simulink model "Controller_implementacion"  (R2026a)
settings: Solver=FixedStepDiscrete  StopTime=inf  FixedStep=Ts  EnableMultiTasking=on
model workspace (MAT data in the model file):
  Ki_SIMC = Simulink.Parameter
  Ki_SIMC.Value = 0.079379
  Ki_SIMC.Complexity = 'real'
  Ki_SIMC.Dimensions = [1 1]
  Ki_SIMC.CoderInfo.StorageClass = 'ExportedGlobal'
  Ki_SIMC.DataType = 'auto'
  Kp_SIMC = Simulink.Parameter
  Kp_SIMC.Value = 7.620337
  Kp_SIMC.Complexity = 'real'
  Kp_SIMC.Dimensions = [1 1]
  Kp_SIMC.CoderInfo.StorageClass = 'ExportedGlobal'
  Kp_SIMC.DataType = 'auto'
  Q_max = Simulink.Parameter
  Q_max.Value = 90
  Q_max.Complexity = 'real'
  Q_max.Dimensions = [1 1]
  Q_max.CoderInfo.StorageClass = 'ExportedGlobal'
  Q_max.DataType = 'single'
  Q_min = Simulink.Parameter
  Q_min.Value = 0
  Q_min.Complexity = 'real'
  Q_min.Dimensions = [1 1]
  Q_min.CoderInfo.StorageClass = 'ExportedGlobal'
  Q_min.DataType = 'single'
  Ts = 1
libraries: slpidlib x1
settings Model: SILPILModeSetting=veronly  ExtModeTrigDuration=2  Creator=jguerrero  LastModifiedBy=jordy
settings HardwareCC: ProdBitPerInt=16.0  ProdBitPerPointer=16.0  ProdBitPerSizeT=16.0  ProdBitPerPtrDiffT=16.0  ProdWordSize=8.0  ProdHWDeviceType=Atmel->AVR
settings ModelReferenceCC: PropagateVarSize=During execution
settings RTWCC: SystemTargetFile=ert.tlc  HardwareBoard=Arduino Leonardo  TLCOptions=-aInlineSetEventsForThisBaseRateFcn=TLC_FALSE -aSuppressMultiTaskScheduler=TLC_FALSE -aRateBasedStepFcn=1  Toolchain=Arduino AVR  BuildConfiguration=Faster Runs  Description=Embedded Coder
settings ERTTargetCC: ExtModeTransport=3.0  ExtModeAutomaticAllocSize=off  ExtModeStaticAllocSize=250.0  CodeInterfacePackaging=Reusable function  SupportContinuousTime=on  SupportVariableSizeSignals=on

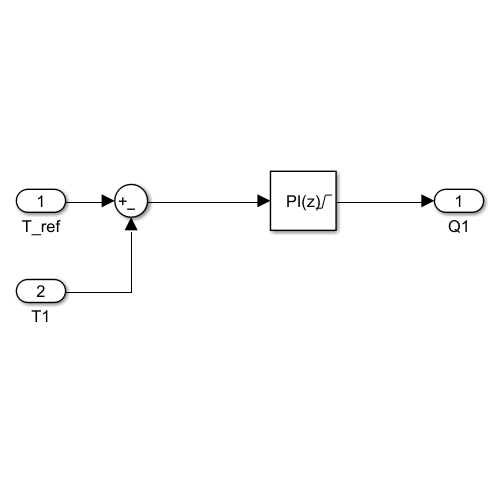
[thumbnail: Simulink's stored preview of the top-level diagram]
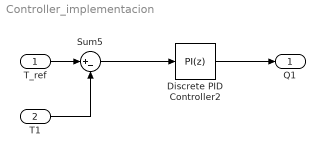
== system Controller_implementacion ==
  T_ref : Inport  OutDataTypeStr=single  PortDimensions=1  SampleTime=[1,0]
  T1 : Inport  Port=2  OutDataTypeStr=single  PortDimensions=1  SampleTime=[1,0]
  Discrete PID Controller2 : slpidlib/PID Controller  Controller=PI  Form=Parallel  TimeDomain=Discrete-time  UseExternalTs=off  SampleTime=Ts  IntegratorMethod=Forward Euler  FilterMethod=Forward Euler  ControllerParametersSource=internal  P=Kp_SIMC  I=Ki_SIMC  UseKiTs=off  D=0  UseExternalDerivativeSource=off  N=100  UseFilter=on  TunerSelectOption=Transfer Function Based (PID Tuner App)  InitialConditionSource=internal  InitialConditionForIntegrator=0  InitialConditionForFilter=0  DifferentiatorICPrevScaledInput=0  ExternalReset=none  TrackingMode=off  Kt=1  LimitOutput=on  SatLimitsSource=internal  UpperSaturationLimit=Q_max  LowerSaturationLimit=Q_min  LinearizeAsGain=off  AntiWindupMode=clamping  Kb=1  LimitIntegrator=off  UpperIntegratorSaturationLimit=inf  LowerIntegratorSaturationLimit=-inf  POutMin=[]  POutMax=[]  IOutMin=[]  IOutMax=[]  DOutMin=[]  DOutMax=[]  NOutMin=[]  NOutMax=[]  SumOutMin=[]  SumOutMax=[]  SaturationOutMin=[]  SaturationOutMax=[]  PParamMin=[]  PParamMax=[]  IParamMin=[]  IParamMax=[]  DParamMin=[]  DParamMax=[]  NParamMin=[]  NParamMax=[]  KbParamMin=[]  KbParamMax=[]  KtParamMin=[]  KtParamMax=[]  KbOutMin=[]  KbOutMax=[]  KtOutMin=[]  KtOutMax=[]  IntegratorOutMin=[]  IntegratorOutMax=[]  FilterOutMin=[]  FilterOutMax=[]  SumI1OutMin=[]  SumI1OutMax=[]  SumI2OutMin=[]  SumI2OutMax=[]  SumI3OutMin=[]  SumI3OutMax=[]  SumI4OutMin=[]  SumI4OutMax=[]  SumDOutMin=[]  SumDOutMax=[]  DifferentiatorOutMin=[]  DifferentiatorOutMax=[]  FilterDiffOutCoefMin=[]  FilterDiffOutCoefMax=[]  ReciprocalOutMin=[]  ReciprocalOutMax=[]  SumDenOutMin=[]  SumDenOutMax=[]  SumNumOutMin=[]  SumNumOutMax=[]  DivideOutMin=[]  DivideOutMax=[]  UdiffTsProdOutMin=[]  UdiffTsProdOutMax=[]  NTsProdOutMin=[]  NTsProdOutMax=[]  UintegralTsProdOutMin=[]  UintegralTsProdOutMax=[]  UngainTsProdOutMin=[]  UngainTsProdOutMax=[]  ClampingZeroOutDataTypeStr=Inherit: Inherit via back propagation  ClampingZeroOutMin=[]  ClampingZeroOutMax=[]  FilterDenConstantOutDataTypeStr=Inherit: Inherit via back propagation  FilterDenConstantOutMin=[]  FilterDenConstantOutMax=[]  PCopyOutDataTypeStr=Inherit: Inherit via back propagation  PCopyOutMin=[]  PCopyOutMax=[]  NCopyOutDataTypeStr=Inherit: Inherit via back propagation  NCopyOutMin=[]  NCopyOutMax=[]  IntegratorContinuousStateAttributes=''  IntegratorStateMustResolveToSignalObject=off  IntegratorRTWStateStorageClass=Auto  FilterContinuousStateAttributes=''  FilterStateMustResolveToSignalObject=off  FilterRTWStateStorageClass=Auto  ParallelPVariant=InternalParameters  IdealPVariant=Disabled  IVariant=InternalParameters  DVariant=Disabled  IntegratorVariant=Discrete  SatVariant=Enabled  AWVariant=DiscClampingParallel  PCopyVariant=Disabled  TRVariant=Disabled  FdbkBlocksVariant=Forward  IdealPFdbkVariant=Disabled  SatFdbkVariant=Disabled  DerivativeFilterVariant=Disabled  NVariant=Disabled  NCopyVariant=Disabled_SignalSpec  FilterICVariant=Disabled  IntegratorICVariant=InternalICs  ExternalResetVariant=Disabled  TRSumVariant=Passthrough  SumFdbkVariant=Disabled  SumVariant=Sum_PI  TsampFilterVariant=InternalTs  TsampNgainVariant=Passthrough  TsampIntegralVariant=Disabled_SignalSpec  ExternalSaturationOutDataTypeStr=Inherit: Same as second input  DerivativeSourceVariant=Disabled  PreIntVariant=InternalPreInt
      settings: LibrarySourceBlock=simulink/Discrete/Discrete PID Controller
  Sum5 : Sum  Inputs=|+-  OutDataTypeStr=single  AccumDataTypeStr=single
  Q1 : Outport  OutMin=0  OutMax=90  OutDataTypeStr=single  PortDimensions=1  SampleTime=[1,0]  LockScale=on
  wires:
  Sum5/1 -> Discrete PID Controller2/1
  T_ref/1 -> Sum5/1
  T1/1 -> Sum5/2
  Discrete PID Controller2/1 -> Q1/1
